simulink model "sf_tetris"  (R2025b)
settings: Solver=ode5  StartTime=0.0  StopTime=inf  FixedStep=1  RelTol=1e-3  EnableMultiTasking=on
settings Model: FPTRunName=Active  ExtModeAutoUpdateStatusClock=off  Creator=The MathWorks, Inc.  LastModifiedBy=The MathWorks, Inc.
settings SolverCC: AlgebraicLoopSolver=TrustRegion
settings DataIOCC: LimitDataPoints=on  SaveFormat=Array  ReturnWorkspaceOutputs=off  SignalLoggingName=sigsOut
settings OptimizationCC: BooleanDataType=off  ReuseModelBlockBuffer=off  ExpressionDepthLimit=2147483647.0  InitFltsAndDblsToZero=on  LifeSpan=inf
settings DebuggingCC: SaveWithParameterizedLinksMsg=none  UnderspecifiedInitializationDetection=Classic  MergeDetectMultiDrivingBlocksExec=none  SignalResolutionControl=TryResolveAllWithWarning  MultiTaskDSMMsg=warning  MultiTaskCondExecSysMsg=none  FcnCallInpInsideContextMsg=warning  UnconnectedInputMsg=warning  UnconnectedOutputMsg=warning  UnconnectedLineMsg=warning  StateNameClashWarn=warning  SFUnexpectedBacktrackingDiag=warning  SFNoUnconditionalDefaultTransitionDiag=warning  SFExecutionAtInitializationDiag=none  ArithmeticOperatorsInVariantConditions=warning
settings HardwareCC: ProdBitPerPointer=32.0  ProdBitPerSizeT=32.0  ProdBitPerPtrDiffT=32.0  ProdLargestAtomicFloat=None  ProdIntDivRoundTo=Undefined  ProdEndianess=Unspecified  ProdWordSize=32.0  ProdHWDeviceType=32-bit Generic  TargetUnknown=on
settings ModelReferenceCC: EnableRefExpFcnMdlSchedulingChecks=on  PropagateSignalLabelsOutOfModel=off
settings SFSimCC: SFSimEcho=off  SimUseLocalCustomCode=off  SimParseCustomCode=off  CustomCodeUndefinedFunction=UseInterfaceOnly
settings RTWCC: RTWUseLocalCustomCode=off  GPUComputeCapability=3.5
settings CodeAppCC: StateflowObjectComments=on
settings GRTTargetCC: TargetFcnLib=ansi_tfl_tmw.mat  TargetLangStandard=C89/C90 (ANSI)  CombineOutputUpdateFcns=off  GRTInterface=on
settings ConfigComp: CovMetricSettings=dcmtr  CovSaveCumulativeToWorkspaceVar=on  CovSaveSingleToWorkspaceVar=on  CovExternalEMLEnable=off  CovSFcnEnable=off

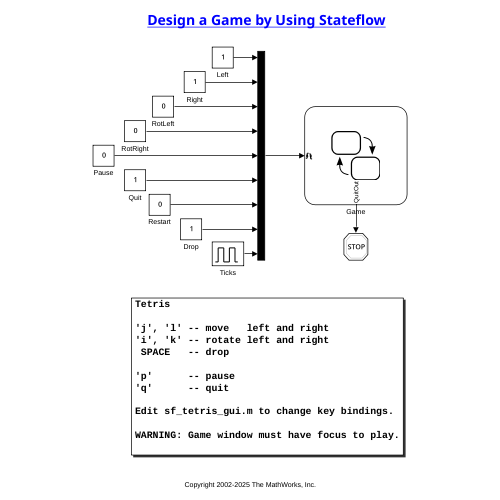
[thumbnail: Simulink's stored preview of the top-level diagram]
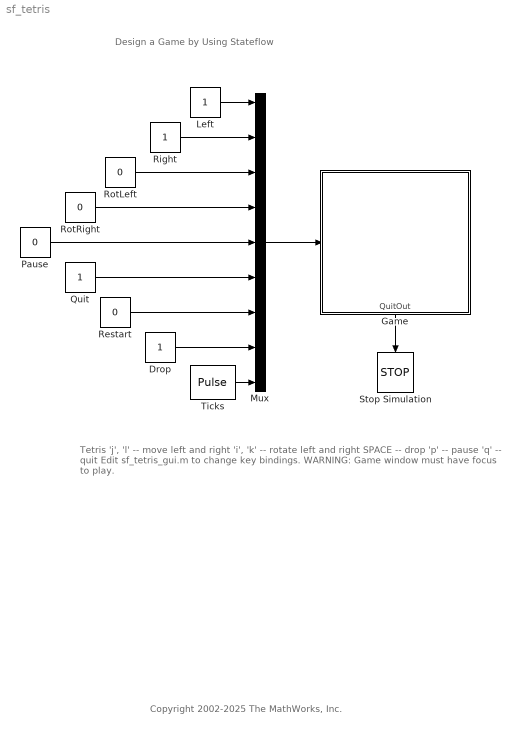
== system sf_tetris ==
  note: Tetris
      |
      | 'j', 'l' -- move   left and right
      | 'i', 'k' -- rotate left and right
      |  SPACE   -- drop
      |
      | 'p'      -- pause
      | 'q'      -- quit
      |
      | Edit sf_tetris_gui.m to change key bindings.
      |
      | WARNING: Game window must have focus to play.
  note: Copyright 2002-2025 The MathWorks, Inc.
  note: Design a Game by Using Stateflow
  Drop : Constant
  Game : Stateflow chart  TreatAsAtomicUnit=on
  Left : Constant
      settings: AttributesFormatString=\n\n
  Mux : Mux  Inputs=9
  Pause : Constant  Value=0
  Quit : Constant
  Restart : Constant  Value=0
  Right : Constant
  RotLeft : Constant  Value=0
  RotRight : Constant  Value=0
  Stop Simulation : Stop
  Ticks : DiscretePulseGenerator  PulseType=Time based  PulseWidth=50
  wires:
  Left/1 -> Mux/1
  Right/1 -> Mux/2
  Mux/1 -> Game/Trigger
  RotRight/1 -> Mux/4
  RotLeft/1 -> Mux/3
  Pause/1 -> Mux/5
  Quit/1 -> Mux/6
  Game/1(QuitOut) -> Stop Simulation/1
  Ticks/1 -> Mux/9
  Restart/1 -> Mux/7
  Drop/1 -> Mux/8

== stateflow chart sf_tetris/Game ==
  state P
  state A
    entry: ml.sf_tetris_gui("paint",level,score);
    exit: t = ml.cputime();
  state Q
    entry:
    ml.sf_tetris_gui('gameover');
    QuitOut;
  state num = clear_rows() [function]
    (default) -> (junction 192) : { y=gridH;
        |   num = 0; }
    (junction 196) -> (junction 197) : { x++; }
    (junction 195) -> (junction 196) [order 1] : [get(x,y)]
    (junction 192) -> (junction 193) [order 1] : [y>=1]
    (junction 193) -> (junction 197) : {x=1;}
    (junction 197) -> (junction 195) [order 1] : [x<=gridW]
    (junction 198) -> (junction 192) : { y--; }
    (junction 192) -> (junction 203) [order 2]
    (junction 197) -> (junction 198) [order 2] : { num++; }
    (junction 195) -> (junction 194) [order 2]
    (junction 194) -> (junction 198) [order 2]
    (junction 194) -> (junction 202) [order 1] : [num!=0]
    (junction 199) -> (junction 198) [order 2]
    (junction 202) -> (junction 199) : { x=1; }
    (junction 199) -> (junction 200) [order 1] : [x<=gridW]
    (junction 201) -> (junction 199) : { x++; }
    (junction 200) -> (junction 201) : { set(x,y+num,get(x,y)); }
  state e = set(x,y,c) [function]
    (default) -> (junction 132)
    (junction 132) -> (junction 136) [order 2] : { e = 1; }
    (junction 132) -> (junction 133) [order 1] : [x>=1 && x<=gridW]
    (junction 133) -> (junction 134) : [y>=1 && y<=gridH]
    (junction 134) -> (junction 135) : { grid[x][y] = c;
        |   ml.sf_tetris_gui("set",y,x,c);
        |  e = 0;
        | }
  state e = show(x,y,s,c) [function]
    (default) -> (junction 155) : { dx = -1;
        |   dy = -1;
        |   i = 0;
        |   e = 0; }
    (junction 155) -> (junction 157) [order 2]
    (junction 155) -> (junction 156) [order 1] : [i<16]
    (junction 156) -> (junction 158) [order 1] : [(s>>i) & 0x1]
    (junction 158) -> (junction 159) : { e+=set(x+dx,y+dy,c); }
    (junction 163) -> (junction 155)
    (junction 156) -> (junction 159) [order 2]
    (junction 159) -> (junction 160) [order 2]
    (junction 159) -> (junction 162) [order 1] : [dx==2]
    (junction 160) -> (junction 161) : {dx++;}
    (junction 162) -> (junction 161) : {dx=-1; dy++;}
    (junction 161) -> (junction 163) : { i++; }
  state r = okay(x,y,s) [function]
    (default) -> (junction 164) : { i = 0;
        |   dx = -1;
        |   dy = -1; }
    (junction 164) -> (junction 149) [order 2]
    (junction 164) -> (junction 147) [order 1] : [i<16]
    (junction 147) -> (junction 145) [order 1] : [(s>>i) & 0x1]
    (junction 145) -> (junction 144) : { r = (get(x+dx,y+dy)==0); }
    (junction 148) -> (junction 164)
    (junction 147) -> (junction 151) [order 2]
    (junction 144) -> (junction 153) [order 1] : [r==0]
    (junction 144) -> (junction 151) [order 2]
    (junction 151) -> (junction 143) [order 2]
    (junction 151) -> (junction 146) [order 1] : [dx==2]
    (junction 146) -> (junction 150) : {dx=-1; dy++;}
    (junction 143) -> (junction 150) : {dx++;}
    (junction 150) -> (junction 148) : { i++; }
  state c = get(x,y) [function]
    (default) -> (junction 137)
    (junction 137) -> (junction 140) [order 3] : { c = 1; }
    (junction 137) -> (junction 176) [order 1] : [y<1] {c = 0; }
    (junction 137) -> (junction 138) [order 2] : [y>=1 && y<=gridH]
    (junction 138) -> (junction 139) : [x>=1 && x<=gridW]
    (junction 139) -> (junction 141) : { c = grid[x][y]; }
  state ns = rot(s,right) [function]
    (default) -> (junction 181) : { i = 0;
        |   ns = 0;
        |   ns |= s & 0xffff0000;
        |   y = 0; }
    (junction 181) -> (junction 187) [order 2]
    (junction 183) -> (junction 181) [order 2] : {y++;}
    (junction 186) -> (junction 183) : {x++; i++;}
    (junction 184) -> (junction 186) [order 2]
    (junction 182) -> (junction 183) : { x = 0; }
    (junction 181) -> (junction 182) [order 1] : [y<4]
    (junction 183) -> (junction 184) [order 1] : [x<4]
    (junction 188) -> (junction 186)
    (junction 184) -> (junction 185) [order 1] : [s>>i & 0x1]
    (junction 185) -> (junction 190) [order 2]
    (junction 185) -> (junction 189) [order 1] : [right]
    (junction 190) -> (junction 191) : { nx = (~y) & 0x3;
        |   ny = x; }
    (junction 189) -> (junction 191) : { nx = y;
        |   ny = (~x) & 0x3; }
    (junction 191) -> (junction 188) : { ns =ns | (1 << (ny*4 + nx)); }
  (junction 178) -> (junction 180)
  (junction 177) -> (junction 178) [order 1] : RotLeft { nS = rot(S,1); }
  (junction 177) -> (junction 285) [order 3]
  (default) -> (junction 213) : {shapes[0] = S1;
      |   shapes[1] = S2;
      |   shapes[2] = S3;
      |   shapes[3] = S4;
      |   shapes[4] = S5;
      |   shapes[5] = S6; }
  (junction 213) -> (junction 210)
  (junction 214) -> (junction 213)
  A -> (junction 213) [order 1] : Restart
  (junction 210) -> A : { ml.sf_tetris_gui("init",gridH,gridW);
      |   X = gridW / 2;
      |   Y = -2;
      |   delay = .1;
      |   clearedRows = 0;
      |   tOld = 0;
      |   t= 0;
      |   S = shapes[0];
      |   grid = 0;
      |   level = 0;
      |   score = 0; }
  (junction 179) -> (junction 180)
  (junction 177) -> (junction 179) [order 2] : RotRight {nS = rot(S,0); }
  (junction 180) -> (junction 168)
  (junction 142) -> (junction 177) [order 3]
  P -> (junction 214) [order 1] : Restart
  (junction 142) -> (junction 166) [order 1] : Left { nX = X - 1;}
  (junction 166) -> (junction 168)
  (junction 168) -> (junction 169) [order 1] : [okay(nX,nY,nS)]
  (junction 142) -> (junction 167) [order 2] : Right { nX = X + 1;}
  (junction 167) -> (junction 168)
  (junction 169) -> (junction 170) : { X = nX;
      |   S = nS; }
  (junction 216) -> (junction 142) [order 3]
  (junction 168) -> (junction 170) [order 2]
  A -> P [order 3] : Pause
  (junction 205) -> A [order 2]
  (junction 205) -> (junction 207) [order 1] : [t-tOld >= delay]
  (junction 207) -> (junction 208)
  P -> A [order 2] : Pause
  (junction 204) -> (junction 205) [order 1] : Ticks
  (junction 208) -> (junction 216) : { offscreen=show(X,Y,S,0);
      |   nX = X;
      |   nY = Y;
      |   nS = S; }
  (junction 216) -> (junction 215) [order 1] : Drop
  (junction 215) -> (junction 170) [order 2] : {Y=nY-1;}
  P -> Q [order 3] : Quit
  (junction 206) -> (junction 208)
  (junction 215) -> (junction 217) [order 1] : [okay(nX,nY,nS)]
  (junction 218) -> (junction 215)
  (junction 216) -> (junction 209) [order 2] : Ticks
  (junction 170) -> (junction 174)
  A -> (junction 204) [order 4]
  (junction 204) -> (junction 206) [order 2]
  (junction 209) -> (junction 165) : { nY = Y + 1;
      |   tOld = t; }
  A -> Q [order 2] : Quit
  (junction 217) -> (junction 218) : {nY++;
      |  score++; }
  (junction 152) -> A : { show(X,Y,S,S>>16); }
  (junction 172) -> Q [order 1] : [offscreen]
  (junction 165) -> (junction 172) [order 2] : { show(X,Y,S,S>>16);
      |   score +=5;
      |   clearedRows += clear_rows();
      |   S = shapes[floor(ml.rand() * 6.0)];
      |   Y = -2;
      |   X = gridW/2; }
  (junction 165) -> (junction 171) [order 1] : [okay(nX,nY,S)]
  (junction 172) -> (junction 211) [order 2]
  (junction 171) -> (junction 154) : { Y = nY; }
  (junction 212) -> (junction 152) : { clearedRows = 0;
      |   delay *= .75;
      |   level++;}
  (junction 211) -> (junction 212) [order 1] : [clearedRows>10]
  (junction 211) -> (junction 152) [order 2]
  (junction 173) -> (junction 152)
  (junction 175) -> (junction 152)
  (junction 154) -> (junction 173)
  (junction 174) -> (junction 175)
  data: num function_output double; x temporary int32; y temporary int32; x function_input int32; y function_input int32; c function_input int32; e function_output int32; x function_input int32; y function_input int32; s function_input int32; dx temporary int32; dy temporary int32; i temporary int32; c function_input int32; e function_output int32; x function_input int32; y function_input int32; r function_output boolean =1; i temporary int32; dy temporary int32; dx temporary int32; s function_input int32; x function_input int32; y function_input int32; c function_output int32; s function_input int32; ns function_output int32; x temporary int32; y temporary int32; i temporary int32; nx temporary int32; ny temporary int32; right function_input boolean; Y local int32 =1; gridW constant int32 =20; gridH constant int32 =60; grid local int8 size=20 60; X local int32 =1; S1 constant int32 =0x202222; nX local int32 =1; nY local int32 =1; shapes local int32 size=6; S2 constant int32 =0x3044c0; S3 constant int32 =0x150360; S4 constant int32 =0x250c60; S local int32; nS local int32; S5 constant int32 =0x3504e0; t local double =1; tOld local double =1; delay local double =1; clearedRows local int32 =1; S6 constant int32 =0x170223; level local int32; score local int32; offscreen local int32 =1
  events: Left input EITHER_EDGE_EVENT; Right input EITHER_EDGE_EVENT; RotLeft input EITHER_EDGE_EVENT; RotRight input EITHER_EDGE_EVENT; Pause input EITHER_EDGE_EVENT; Quit input EITHER_EDGE_EVENT; Restart input EITHER_EDGE_EVENT; Drop input EITHER_EDGE_EVENT; Ticks input EITHER_EDGE_EVENT; QuitOut output EITHER_EDGE_EVENT
